simulink subsystem "Subsys_GFormConv_Control"  (R2023b)
settings: Solver=VariableStepAuto  StartTime=0.0  StopTime=10.0  RelTol=1e-3
model mask{S_n=2e6, f_n=50, V_n_phph=690, V_n_grid_phph=20e3, V_n_dc=1380, RL_filter_conv_pu=[ 0.0001 0.05097 ], RC_filter_pu=[ 0.06875 0.04569 ], outputSignal=0, f_sw=5000, sendInfoMessages=0, T_s_ctrl=1e-4, T_s_PWM_meas=1e-4, datatype='double', meas_signals=0, meas_noise_filter=1, f_cutoff_meas=2500, f_cutoff_posseq=20, prot_variant=1, v_dc_max=1.2, v_ac_max=1.1, t_ac_max=0.1, v_ac_maxmax=1.25, t_ac_maxmax=0.1, v_ac_min=0.8, t_ac_min=3, v_ac_minmin=0.45, t_ac_minmin=0.3, f_ac_max=51.5, t_f_ac_max=0.1, f_ac_maxmax=52.5, t_f_ac_maxmax=10, f_ac_min=47.5, t_f_ac_min=0.1, i_ac_max=1.25, OuterCtrlStrategy=0, OuterCtrl_Droop_kP=0.05, OuterCtrl_Droop_kQ=0.1, OuterCtrl_Droop_TQ=0.2, OuterCtrl_ZDroop_kf=0.05, OuterCtrl_ZDroop_kV=0.1, OuterCtrl_ZDroop_kR=0, OuterCtrl_ZDroop_kX=1, OuterCtrl_ZDroop_TV=2, OuterCtrl_Dual_Kp=0.01, OuterCtrl_Dual_Kd=1e-4, OuterCtrl_Dual_kQ=0.1, OuterCtrl_Dual_TQ=0.2, OuterCtrl_VSM_H=0.1, OuterCtrl_VSM_Kd=40, OuterCtrl_VSM_K=20, OuterCtrl_VSM_kQ=0.1, OuterCtrl_VSM_TQ=0.2, L_virt=0, active_damping=1, R_virt_pu=0.2, InnerCtrl_K_p_v_cap=0.8, InnerCtrl_K_i_v_cap=0.5, InnerCtrl_K_p_i_conv=3.3, InnerCtrl_K_i_i_conv=16.5, InnerCtrl_C_ff_v_cap_ctrl=0, InnerCtrl_C_ff_i_conv_ctrl=0, InnerCtrl_K_ff_i=1, InnerCtrl_K_ff_v=1, InnerCtrl_i_conv_max=1, InnerCtrl_v_conv_max=1.3, InnerCtrl_i_lim_type=0}
  mask prompts: S_n "Nominal apparent power [VA]"; f_n "Nominal frequency [Hz]"; V_n_phph "Nominal converter voltage (rms, phase-to-phase) [V]"; V_n_grid_phph "Nominal grid voltage (rms, phase-to-phase) [V]"; V_n_dc "Nominal DC-link voltage [V]"; RL_filter_conv_pu "Impedance of converter-side inductance [ R L ] (pu)"; RC_filter_pu "Impedance of filter capacitor [ R C ] (pu)"; outputSignal "Output signal type (2 = duty cycle (imperix), 1 = switching pulses, 0 = voltage reference (average model))"; f_sw "Switching frequency [Hz]"; sendInfoMessages "Send info messages (1 = enabled, 0 = disabled)"; T_s_ctrl "Controller sample time [s]"; T_s_PWM_meas "PWM and measurements sample time [s]"; datatype "Signal data type"; meas_signals "Measured signals (0 = all signals (tDMSquared simulation), 1 = reduced signals (imperix hardware))"; meas_noise_filter "Low pass to filter measurement noise (1 = enabled, 0 = disabled)"; f_cutoff_meas "Cutoff frequency of low pass filter (measurement noise) [Hz]"; f_cutoff_posseq "Cutoff frequency of low pass filter (positive sequence calculation) [Hz]"; prot_variant "Protection Variant (1 = hardware protection, 2 = tDMSquared warnings only, 3 = deactivated)"; v_dc_max "Maximum DC-link voltage [% nom. value]"; v_ac_max "Maximum AC voltage [% nom. value]"; t_ac_max "Maximum AC voltage timing [s]"; v_ac_maxmax "Upper Maximum AC voltage [% nom. value]"; t_ac_maxmax "Upper Maximum AC voltage timing [s]"; v_ac_min "Upper Minimum AC voltage [% nom. value]"; t_ac_min "Upper Minimum AC voltage timing [s]"; v_ac_minmin "Lower Minimum AC voltage [% nom. value]"; t_ac_minmin "Lower Minimum AC voltage timing [s]"; f_ac_max "Maximum AC frequency [Hz]"; t_f_ac_max "Maximum AC frequency timing [s]"; f_ac_maxmax "Upper Maximum AC frequency [Hz]"; t_f_ac_maxmax "Upper Maximum AC frequency timing [s]"; f_ac_min "Minimum AC frequency [Hz]"; t_f_ac_min "Minimum AC frequency timing [s]"; i_ac_max "Maximum AC current [% nom. value]"; OuterCtrlStrategy "Outer Control Strategy*"; OuterCtrl_Droop_kP "Droop constant kP (df[pu]/dP[pu])"; OuterCtrl_Droop_kQ "Droop constant kQ (dV[pu]/dQ[pu])"; OuterCtrl_Droop_TQ "PT1 time constant QV-loop [s]"; OuterCtrl_ZDroop_kf "Droop constant kf (df/(dP+dQ))"; OuterCtrl_ZDroop_kV "Droop constant kV (dV/(dP+dQ))"; OuterCtrl_ZDroop_kR "R/Z-ratio"; OuterCtrl_ZDroop_kX "X/Z-ratio"; OuterCtrl_ZDroop_TV "PT1 time constant voltage loop [s]"; OuterCtrl_Dual_Kp "Proportional gain [pu]"; OuterCtrl_Dual_Kd "Derivative gain [pu]"; OuterCtrl_Dual_kQ "Droop constant kQ (dV/dQ)"; OuterCtrl_Dual_TQ "PT1 time constant QV-loop T_Q [s]"; OuterCtrl_VSM_H "Virtual inertia [s]"; OuterCtrl_VSM_Kd "Damping constant K_d [pu]"; OuterCtrl_VSM_K "Droop constant K (dT/df) [pu]"; OuterCtrl_VSM_kQ "Droop constant kQ (dV/dQ)"; OuterCtrl_VSM_TQ "PT1 time constant QV-loop T_Q [s]"; L_virt "Virtual output inductance [pu]"; active_damping "Active Damping (1 = enabled, 0 = disabled)"; R_virt_pu "Virtual resistor for active damping (in series with converter-side inductor) [pu]"; InnerCtrl_K_p_v_cap "Voltage controller proportional gain [pu]"; InnerCtrl_K_i_v_cap "Voltage controller integral gain [pu]"; InnerCtrl_K_p_i_conv "Current controller proportional gain [pu]"; InnerCtrl_K_i_i_conv "Current controller integral gain [pu]"; InnerCtrl_C_ff_v_cap_ctrl "Command-feed-forward (voltage controller) (0 = disabled, 1 = enabled)"; InnerCtrl_C_ff_i_conv_ctrl "Command-feed-forward (current controller) (0 = disabled, 1 = enabled)"; InnerCtrl_K_ff_i "Current-feed-forward (voltage controller) (0 = disabled, 1 = enabled)"; InnerCtrl_K_ff_v "Voltage-feed-forward (current controller) (0 = disabled, 1 = enabled)"; InnerCtrl_i_conv_max "Converter current maximum value (limit) [pu]"; InnerCtrl_v_conv_max "Converter voltage maximum value (limit) [pu]"; InnerCtrl_i_lim_type "Coordinate system of current setpoint limiter (0 = dq, 1 = abc)"
libraries: eeTransforms x2, simulink x2, eePwmGeneratorTwoLevel x1
settings Model: Creator=winkens  LastModifiedBy=a.och
settings SolverCC: AlgebraicLoopSolver=TrustRegion
settings OptimizationCC: ReuseModelBlockBuffer=off
settings DebuggingCC: UnconnectedInputMsg=warning  UnconnectedOutputMsg=warning  UnconnectedLineMsg=warning
settings ModelReferenceCC: EnableRefExpFcnMdlSchedulingChecks=on
settings RTWCC: DLArmComputeVersion=19.05

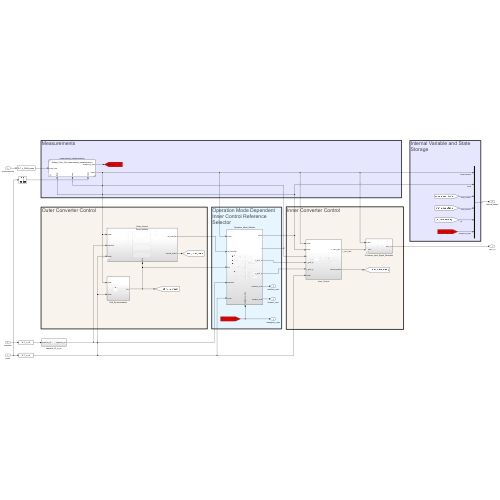
[thumbnail: Simulink's stored preview of the top-level diagram]
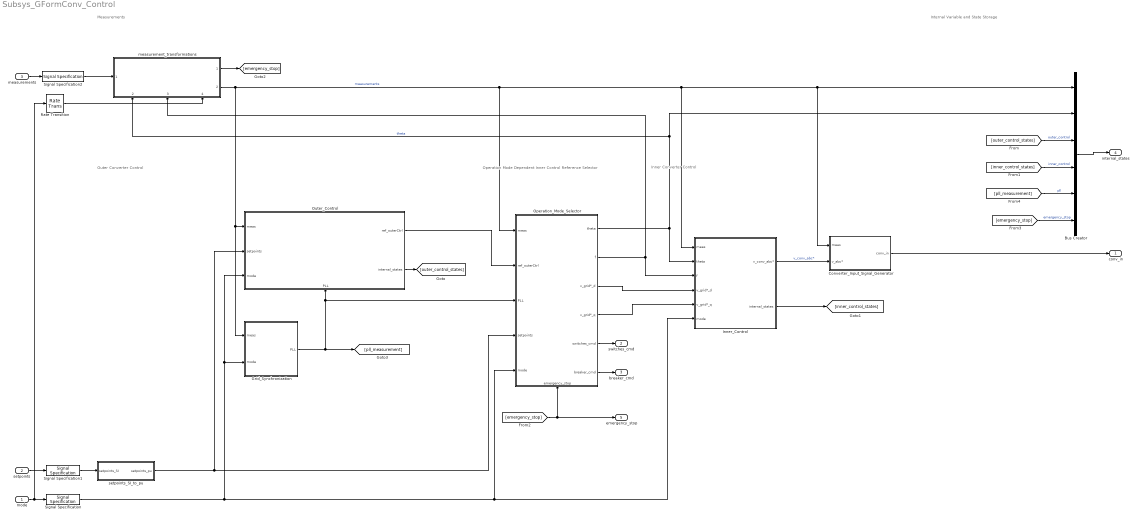
== system Subsys_GFormConv_Control ==
  note: Operation Mode Dependent
      | Inner Control Reference
      | Selector
  note: Outer Converter Control
  note: Internal Variable and State
      | Storage
  note: Inner Converter Control
  note: Measurements
  mode : Inport
  setpoints : Inport  Port=2
  measurements : Inport  Port=3
  Bus Creator : BusCreator  Inputs=6
  Converter_Input_Signal_Generator : Subsystem  Variant=on
  Grid_Synchronization : Subsystem
  Inner_Control : Subsystem
  Operation_Mode_Selector : Subsystem
      settings: PortSchema="{\"entries\":[{\"content\":{\"sides\":[{\"content\":{\"connectorIds\":[\"In1\",\"In2\",\"In3\",\"In4\",\"In5\"]},\"type\":\"ConnectorPlacement.EquallySpacedRectSide\",\"uuid\":\"66bc241c-88d5-476d-bdbe-e179bef52087\"},{\"content\":{\"connectorIds\":[\"Out1\",\"Out2\",\"Out3\",\"Out4\",\"Out5\",\"Out6\"],\"side\":\"RIGHT\"},\"type\":\"ConnectorPlacement.EquallySpacedRectSide\",\"uuid\":\"318c79a0-3cc7-4e7d-956b-e38d7c55976e\"},{\"content\":{\"connectorIds\":[],\"side\":\"TOP\"},\"type\":\"ConnectorPlacement.EquallySpacedRectSide\",\"uuid\":\"dd042cf5-83ab-40ed-a1fe-bca14fe85d10\"},{\"content\":{\"connectorIds\":[\"In6\"],\"side\":\"BOTTOM\"},\"type\":\"ConnectorPlacement.EquallySpacedRectSide\",\"uuid\":\"10d73b36-3b70-4044-8718-174bd2d17802\"},{\"content\":{\"connectorIds\":[],\"side\":\"HIDDEN\"},\"type\":\"ConnectorPlacement.EquallySpacedRectSide\",\"uuid\":\"4c9d2e62-9083-4dbd-9c06-7f98e71bb5f3\"}]},\"type\":\"ConnectorPlacement.EquallySpacedConnector\",\"uuid\":\"f943bfea-1324-4575-985b-fb99fa51a3d8\"}],\"packageUris\":[\"http://schema.mathworks.com/mf0/Connector/R2020b\"],\"version\":\"1.0\"}"
  Outer_Control : Subsystem  Variant=on
      settings: PortSchema="{\"entries\":[{\"content\":{\"sides\":[{\"content\":{\"connectorIds\":[\"In1\",\"In2\",\"In3\"]},\"type\":\"ConnectorPlacement.EquallySpacedRectSide\",\"uuid\":\"253b05e4-806f-4dc0-80d3-d592634157a9\"},{\"content\":{\"connectorIds\":[\"Out1\",\"Out2\"],\"side\":\"RIGHT\"},\"type\":\"ConnectorPlacement.EquallySpacedRectSide\",\"uuid\":\"c3b70f7b-68db-4cd5-a2c2-c4f65ef550a5\"},{\"content\":{\"connectorIds\":[],\"side\":\"TOP\"},\"type\":\"ConnectorPlacement.EquallySpacedRectSide\",\"uuid\":\"830f2dd0-f758-4d50-8b34-5845389ea785\"},{\"content\":{\"connectorIds\":[\"In4\"],\"side\":\"BOTTOM\"},\"type\":\"ConnectorPlacement.EquallySpacedRectSide\",\"uuid\":\"b9313e94-082c-4f29-831f-6939b42f2aae\"},{\"content\":{\"connectorIds\":[],\"side\":\"HIDDEN\"},\"type\":\"ConnectorPlacement.EquallySpacedRectSide\",\"uuid\":\"42ff5aed-1d40-40fc-b6bc-8c88d6312836\"}]},\"type\":\"ConnectorPlacement.EquallySpacedConnector\",\"uuid\":\"adca5aff-478b-45b4-94a3-86875e004fa1\"}],\"packageUris\":[\"http://schema.mathworks.com/mf0/Connector/R2020b\"],\"version\":\"1.0\"}"
  Rate Transition : RateTransition  OutPortSampleTime=T_s_PWM_meas
  Signal Specification : SignalSpecification  SampleTime=T_s_ctrl
  Signal Specification1 : SignalSpecification  SampleTime=T_s_ctrl
  Signal Specification2 : SignalSpecification  SampleTime=T_s_PWM_meas
  measurement_transformations : Subsystem  ReferencedSubsystem=Subsys_Conv_Ctrl_measurement_transformations  S_n=S_n  f_n=f_n  V_n_phph=V_n_phph  V_n_grid_phph=V_n_grid_phph  V_n_dc=V_n_dc  meas_signals=meas_signals  meas_noise_filter=meas_noise_filter  f_cutoff_lowpass=f_cutoff_meas  posseq_calc=0  f_cutoff_posseq=f_cutoff_posseq  prot_variant=prot_variant  v_dc_max=v_dc_max  v_ac_max=v_ac_max  t_ac_max=t_ac_max  v_ac_maxmax=v_ac_maxmax  t_ac_maxmax=t_ac_maxmax  v_ac_min=v_ac_min  t_ac_min=t_ac_min  v_ac_minmin=v_ac_minmin  t_ac_minmin=t_ac_minmin  f_ac_max=f_ac_max  t_f_ac_max=t_f_ac_max  f_ac_maxmax=f_ac_maxmax  t_f_ac_maxmax=t_f_ac_maxmax  f_ac_min=f_ac_min  t_f_ac_min=t_f_ac_min  i_ac_max=i_ac_max  T_s_ctrl=T_s_ctrl  T_s_PWM_meas=T_s_PWM_meas  datatype=datatype
      settings: PortSchema="{\"entries\":[{\"content\":{\"sides\":[{\"content\":{\"connectorIds\":[\"In1\"]},\"type\":\"ConnectorPlacement.EquallySpacedRectSide\",\"uuid\":\"ec41b0e2-5656-4860-9e39-a664af2bd5a5\"},{\"content\":{\"connectorIds\":[\"Out1\",\"Out2\"],\"side\":\"RIGHT\"},\"type\":\"ConnectorPlacement.EquallySpacedRectSide\",\"uuid\":\"80e01e50-a82e-48c2-876d-2e84cdeaf8f0\"},{\"content\":{\"side\":\"TOP\"},\"type\":\"ConnectorPlacement.EquallySpacedRectSide\",\"uuid\":\"663ee62b-f6cc-4583-9600-029eedfe0a7c\"},{\"content\":{\"connectorIds\":[\"In2\",\"In3\",\"In4\"],\"side\":\"BOTTOM\"},\"type\":\"ConnectorPlacement.EquallySpacedRectSide\",\"uuid\":\"c2907c22-84a2-4ef4-81a7-f2773dfe6a2a\"},{\"content\":{\"side\":\"HIDDEN\"},\"type\":\"ConnectorPlacement.EquallySpacedRectSide\",\"uuid\":\"af4de394-2758-4e50-9887-b7deaef1f38c\"}]},\"type\":\"ConnectorPlacement.EquallySpacedConnector\",\"uuid\":\"1362d2e6-f83a-419a-8b0e-95b4449907fb\"}],\"packageUris\":[\"http://schema.mathworks.com/mf0/Connector/R2020b\"],\"version\":\"1.0\"}"
  setpoints_SI_to_pu : Subsystem
  conv_in : Outport
  switches_cmd : Outport  Port=2
  breaker_cmd : Outport  Port=3
  internal_states : Outport  Port=4
  emergency_stop : Outport  Port=5
  wires:
  Rate Transition/1 -> measurement_transformations/4
  Operation_Mode_Selector/2(f) -> measurement_transformations/3, Inner_Control/3(f)
  setpoints/1 -> Signal Specification1/1
  Inner_Control/1(v_conv_abc*) -> Converter_Input_Signal_Generator/2(v_abc*)  "v_conv_abc*"
  Inner_Control/2(internal_states) -> [inner_control_states]
  [outer_control_states] -> Bus Creator/3  "outer_control"
  [inner_control_states] -> Bus Creator/4  "inner_control"
  Bus Creator/1 -> internal_states/1
  Outer_Control/2(internal_states) -> [outer_control_states]
  mode/1 -> Signal Specification/1, Rate Transition/1
  Operation_Mode_Selector/3(v_grid*_d) -> Inner_Control/4(v_grid*_d)
  Operation_Mode_Selector/1(theta) -> Inner_Control/2(theta), Bus Creator/2, measurement_transformations/2  "theta"
  Outer_Control/1(ref_outerCtrl) -> Operation_Mode_Selector/2(ref_outerCtrl)
  Operation_Mode_Selector/5(switches_cmd) -> switches_cmd/1
  Operation_Mode_Selector/6(breaker_cmd) -> breaker_cmd/1
  Converter_Input_Signal_Generator/1(conv_in) -> conv_in/1
  setpoints_SI_to_pu/1(setpoints_pu) -> Outer_Control/2(setpoints), Operation_Mode_Selector/4(setpoints)
  Grid_Synchronization/1(PLL) -> [pll_measurement], Operation_Mode_Selector/3(PLL), Outer_Control/4(PLL)
  measurement_transformations/2 -> Outer_Control/1(meas), Grid_Synchronization/1(meas), Converter_Input_Signal_Generator/1(meas), Bus Creator/1, Inner_Control/1(meas), Operation_Mode_Selector/1(meas)  "measurements"
  measurements/1 -> Signal Specification2/1
  measurement_transformations/1 -> [emergency_stop]
  [emergency_stop] -> emergency_stop/1, Operation_Mode_Selector/6(emergency_stop)
  Signal Specification/1 -> Inner_Control/6(mode), Operation_Mode_Selector/5(mode), Grid_Synchronization/2(mode), Outer_Control/3(mode)
  Signal Specification1/1 -> setpoints_SI_to_pu/1(setpoints_SI)
  Signal Specification2/1 -> measurement_transformations/1
  Operation_Mode_Selector/4(v_grid*_q) -> Inner_Control/5(v_grid*_q)
  [emergency_stop] -> Bus Creator/6  "emergency_stop"
  [pll_measurement] -> Bus Creator/5  "pll"

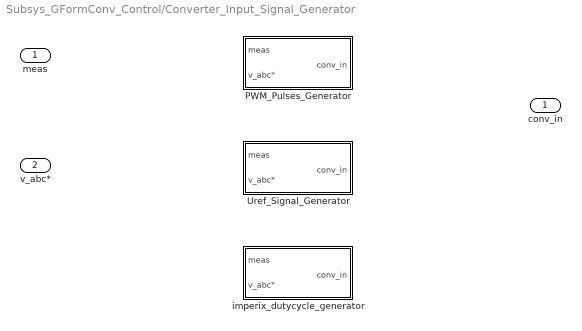
== system Subsys_GFormConv_Control/Converter_Input_Signal_Generator ==
  meas : Inport
  v_abc* : Inport  Port=2
  PWM_Pulses_Generator : Subsystem  VariantControl=outputSignal == 1
  Uref_Signal_Generator : Subsystem  VariantControl=(default)
  imperix_dutycycle_generator : Subsystem  VariantControl=outputSignal == 2
  conv_in : Outport

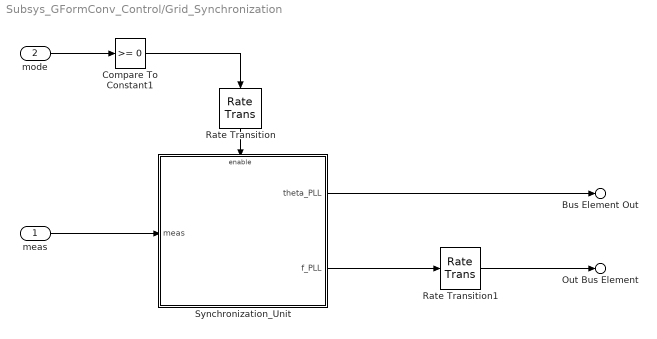
== system Subsys_GFormConv_Control/Grid_Synchronization ==
  meas : Inport
  mode : Inport  Port=2
  Compare To Constant1 : simulink/Logic and Bit Operations/Compare To Constant  relop=>=  const=0  OutDataTypeStr=boolean
  Rate Transition : RateTransition  Deterministic=off  OutPortSampleTime=T_s_PWM_meas
  Rate Transition1 : RateTransition  Deterministic=off  OutPortSampleTime=T_s_ctrl
  Synchronization_Unit : Subsystem
  Bus Element Out : Outport  PortName=PLL  Element=theta_PLL
  Out Bus Element : Outport  PortName=PLL  Element=f_PLL
  wires:
  meas/1 -> Synchronization_Unit/1(meas)
  mode/1 -> Compare To Constant1/1
  Compare To Constant1/1 -> Rate Transition/1
  Synchronization_Unit/1(theta_PLL) -> Bus Element Out/1
  Synchronization_Unit/2(f_PLL) -> Rate Transition1/1
  Rate Transition/1 -> Synchronization_Unit/Enable
  Rate Transition1/1 -> Out Bus Element/1

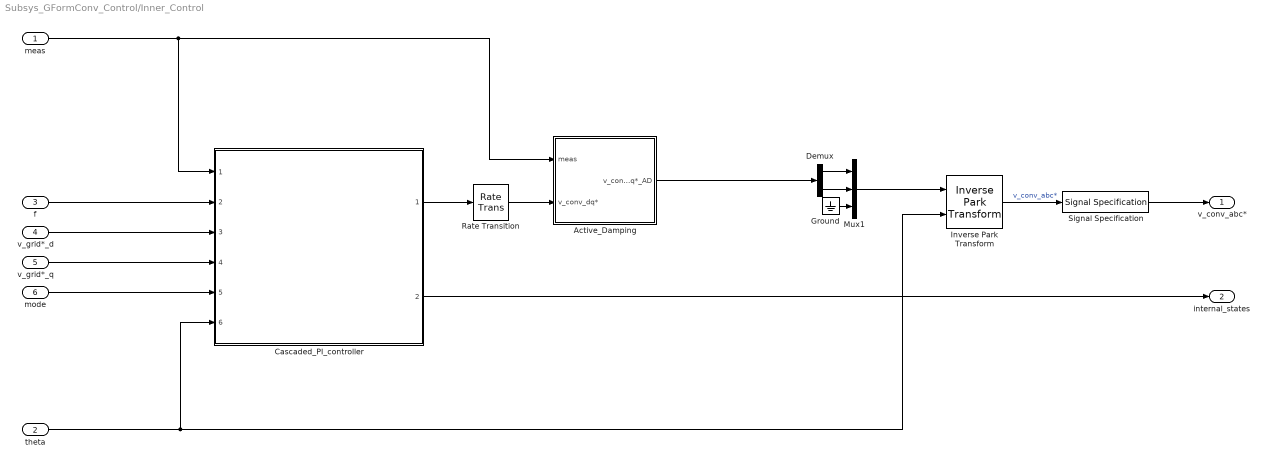
== system Subsys_GFormConv_Control/Inner_Control ==
  meas : Inport
  theta : Inport  Port=2  PortDimensions=1
  f : Inport  Port=3  PortDimensions=1
  v_grid*_d : Inport  Port=4  PortDimensions=1
  v_grid*_q : Inport  Port=5  PortDimensions=1
  mode : Inport  Port=6  PortDimensions=1
  Active_Damping : Subsystem  Variant=on  VariantControl=Choice
  Cascaded_PI_controller : Subsystem  ReferencedSubsystem=Subsys_GFormConv_InnerCtrl_cascadedPI  f_n=f_n  L_filter_conv_pu=RL_filter_conv_pu  C_filter_pu=RC_filter_pu  send_info_messages=sendInfoMessages  K_p_V_cap_controller=InnerCtrl_K_p_v_cap  K_i_V_cap_controller=InnerCtrl_K_i_v_cap  K_p_I_conv_controller=InnerCtrl_K_p_i_conv  K_i_I_conv_controller=InnerCtrl_K_i_i_conv  Cff_V_cap_ctrl=InnerCtrl_C_ff_v_cap_ctrl  Cff_I_conv_ctrl=InnerCtrl_C_ff_i_conv_ctrl  K_ff_I_grid=InnerCtrl_K_ff_i  K_ff_V_cap=InnerCtrl_K_ff_v  i_conv_limit=InnerCtrl_i_conv_max  v_conv_limit=InnerCtrl_v_conv_max  i_lim_type=InnerCtrl_i_lim_type  T_s_ctrl=T_s_ctrl  T_s_PWM_meas=T_s_PWM_meas  datatype=datatype
  Demux : Demux  Outputs=2
  Ground : Ground
  Inverse Park Transform : eeTransforms/Inverse Park Transform  AxisAlignment=D-axis  PowerInvariant=off
  Mux1 : Mux  Inputs=3
  Rate Transition : RateTransition  Deterministic=off  OutPortSampleTime=T_s_PWM_meas
  Signal Specification : SignalSpecification  SampleTime=T_s_PWM_meas
  v_conv_abc* : Outport  PortDimensions=3
  internal_states : Outport  Port=2
  wires:
  meas/1 -> Active_Damping/1(meas), Cascaded_PI_controller/1
  f/1 -> Cascaded_PI_controller/2
  v_grid*_d/1 -> Cascaded_PI_controller/3
  mode/1 -> Cascaded_PI_controller/5
  Cascaded_PI_controller/2 -> internal_states/1
  Mux1/1 -> Inverse Park Transform/1
  Ground/1 -> Mux1/3
  Demux/2 -> Mux1/2
  Demux/1 -> Mux1/1
  theta/1 -> Cascaded_PI_controller/6, Inverse Park Transform/2
  Cascaded_PI_controller/1 -> Rate Transition/1
  Inverse Park Transform/1 -> Signal Specification/1  "v_conv_abc*"
  Active_Damping/1(v_conv_dq*_AD) -> Demux/1
  Signal Specification/1 -> v_conv_abc*/1
  Rate Transition/1 -> Active_Damping/2(v_conv_dq*)
  v_grid*_q/1 -> Cascaded_PI_controller/4

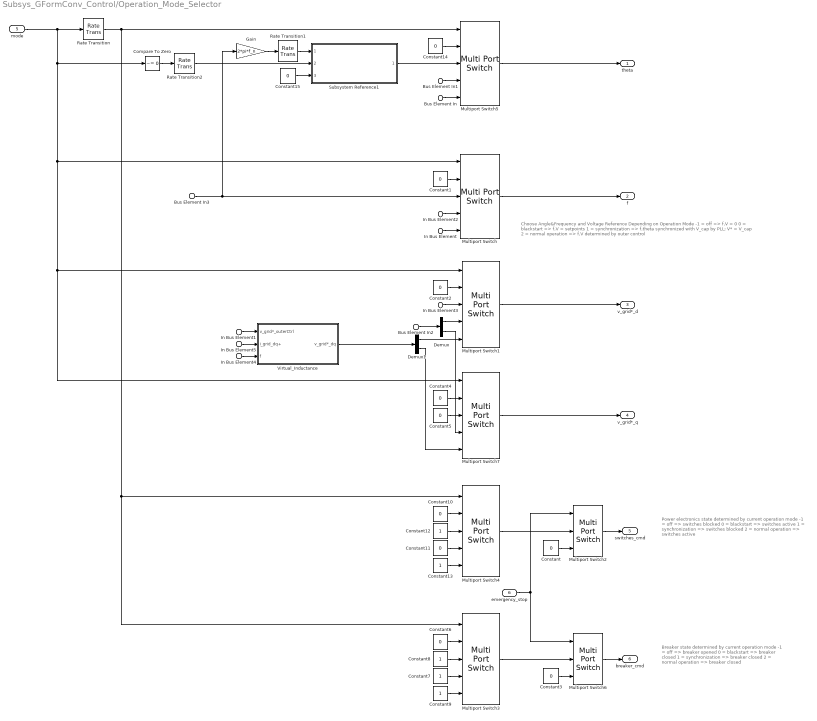
== system Subsys_GFormConv_Control/Operation_Mode_Selector ==
  note: Choose Angle&Frequency and Voltage Reference Depending on Operation Mode
      | -1 = off => f,V = 0
      | 0 = blackstart => f,V = setpoints
      | 1 = synchronization => f,theta synchronized with V_cap by PLL; V* = V_cap
      | 2 = normal operation => f,V determined by outer control
  note: Breaker state determined by current operation mode
      | -1 = off => breaker opened
      | 0  = blackstart => breaker closed
      | 1  = synchronization => breaker closed
      | 2  = normal operation => breaker closed
  note: Power electronics state determined by current operation mode
      | -1 = off => switches blocked
      | 0  = blackstart => switches active
      | 1  = synchronization => switches blocked
      | 2  = normal operation => switches active
  Bus Element In2 : Inport  PortName=meas  Element=dq+.v_cap_dq+
  In Bus Element5 : Inport  PortName=meas  Element=dq+.i_grid_dq+
  Bus Element In : Inport  Port=2  PortName=ref_outerCtrl  Element=theta
  In Bus Element : Inport  Port=2  PortName=ref_outerCtrl  Element=f
  In Bus Element4 : Inport  Port=2  PortName=ref_outerCtrl  Element=f
  In Bus Element1 : Inport  Port=2  PortName=ref_outerCtrl  Element=v_grid*
  Bus Element In1 : Inport  Port=3  PortName=PLL  Element=theta_PLL
  In Bus Element2 : Inport  Port=3  PortName=PLL  Element=f_PLL
  Bus Element In3 : Inport  Port=4  PortName=setpoints  Element=f_set_pu
  In Bus Element3 : Inport  Port=4  PortName=setpoints  Element=v_set
  mode : Inport  Port=5
  emergency_stop : Inport  Port=6
  Compare To Zero : simulink/Logic and Bit Operations/Compare To Zero  relop=~=  OutDataTypeStr=boolean
  Constant{,3,6,10..11} (5 alike) : Constant  Value=0  OutDataTypeStr=boolean
  Constant{1..2,4..5,14} (5 alike) : Constant  Value=0  OutDataTypeStr=datatype
  Constant{7..9,12..13} (5 alike) : Constant  OutDataTypeStr=boolean
  Constant15 : Constant  Value=0
  Demux : Demux  Outputs=2
  Demux1 : Demux  Outputs=2
  Gain : Gain  Gain=2*pi*f_n
  Multiport Switch{,1,3..5,7} (6 alike) : MultiPortSwitch  DataPortOrder=Specify indices  DataPortIndices={-1,0,1,2}  SaturateOnIntegerOverflow=off  InputSameDT=off
  Multiport Switch2 : MultiPortSwitch  DataPortOrder=Specify indices  DataPortIndices={0,1}  SaturateOnIntegerOverflow=off  InputSameDT=off
  Multiport Switch6 : MultiPortSwitch  DataPortOrder=Specify indices  DataPortIndices={0,1}  SaturateOnIntegerOverflow=off  InputSameDT=off
  Rate Transition : RateTransition  Deterministic=off  OutPortSampleTime=T_s_PWM_meas
  Rate Transition1 : RateTransition  Deterministic=off  OutPortSampleTime=T_s_PWM_meas
  Rate Transition2 : RateTransition  Deterministic=off  OutPortSampleTime=T_s_PWM_meas
  Subsystem Reference1 : Subsystem  ReferencedSubsystem=Integrator_discrete_wrapped_state  WrappedStateUpperValue=2*pi  WrappedStateLowerValue=0  x_0=0  T_s=T_s_PWM_meas
  Virtual_Inductance : Subsystem
  theta : Outport
  f : Outport  Port=2
  v_grid*_d : Outport  Port=3
  v_grid*_q : Outport  Port=4
  switches_cmd : Outport  Port=5
  breaker_cmd : Outport  Port=6
  wires:
  Gain/1 -> Rate Transition1/1
  Bus Element In1/1 -> Multiport Switch5/4
  In Bus Element2/1 -> Multiport Switch/4
  Demux/1 -> Multiport Switch1/4
  In Bus Element3/1 -> Multiport Switch1/3
  Bus Element In3/1 -> Multiport Switch/3, Gain/1
  Constant2/1 -> Multiport Switch1/2
  In Bus Element/1 -> Multiport Switch/5
  Constant1/1 -> Multiport Switch/2
  Multiport Switch1/1 -> v_grid*_d/1
  Multiport Switch/1 -> f/1
  Constant7/1 -> Multiport Switch3/4
  Constant6/1 -> Multiport Switch3/2
  Constant10/1 -> Multiport Switch4/2
  Constant8/1 -> Multiport Switch3/3
  Constant12/1 -> Multiport Switch4/3
  Constant13/1 -> Multiport Switch4/5
  Constant9/1 -> Multiport Switch3/5
  Constant11/1 -> Multiport Switch4/4
  mode/1 -> Rate Transition/1, Compare To Zero/1, Multiport Switch/1, Multiport Switch7/1, Multiport Switch1/1
  Bus Element In/1 -> Multiport Switch5/5
  Demux/2 -> Multiport Switch7/4
  Multiport Switch5/1 -> theta/1
  Constant14/1 -> Multiport Switch5/2
  Constant15/1 -> Subsystem Reference1/3
  Compare To Zero/1 -> Rate Transition2/1
  Subsystem Reference1/1 -> Multiport Switch5/3
  emergency_stop/1 -> Multiport Switch6/1, Multiport Switch2/1
  Multiport Switch2/1 -> switches_cmd/1
  Multiport Switch6/1 -> breaker_cmd/1
  Multiport Switch3/1 -> Multiport Switch6/2
  Multiport Switch4/1 -> Multiport Switch2/2
  Constant/1 -> Multiport Switch2/3
  Constant3/1 -> Multiport Switch6/3
  Bus Element In2/1 -> Demux/1
  Rate Transition/1 -> Multiport Switch3/1, Multiport Switch4/1, Multiport Switch5/1
  Rate Transition1/1 -> Subsystem Reference1/1
  Rate Transition2/1 -> Subsystem Reference1/2
  Multiport Switch7/1 -> v_grid*_q/1
  Constant5/1 -> Multiport Switch7/3
  Constant4/1 -> Multiport Switch7/2
  Demux1/1 -> Multiport Switch1/5
  Virtual_Inductance/1(v_grid*_dq) -> Demux1/1
  Demux1/2 -> Multiport Switch7/5
  In Bus Element1/1 -> Virtual_Inductance/1(v_grid*_outerCtrl)
  In Bus Element4/1 -> Virtual_Inductance/3(f)
  In Bus Element5/1 -> Virtual_Inductance/2(i_grid_dq+)

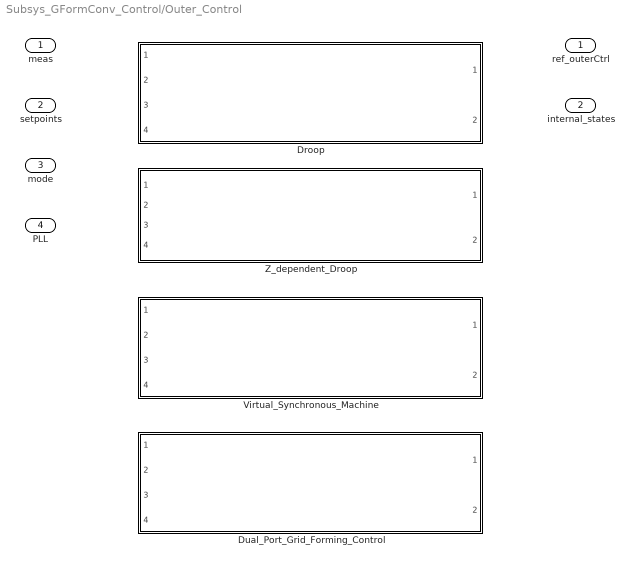
== system Subsys_GFormConv_Control/Outer_Control ==
  meas : Inport
  setpoints : Inport  Port=2
  mode : Inport  Port=3
  PLL : Inport  Port=4
  Droop : Subsystem  VariantControl=(default)  ReferencedSubsystem=Subsys_GFormConv_OuterCtrl_Droop  f_n=f_n  s_droop_Pf=OuterCtrl_Droop_kP  s_droop_QV=OuterCtrl_Droop_kQ  T_Q=OuterCtrl_Droop_TQ  T_s_ctrl=T_s_ctrl  T_s_PWM_meas=T_s_PWM_meas
  Dual_Port_Grid_Forming_Control : Subsystem  VariantControl=OuterCtrlStrategy == 3  ReferencedSubsystem=Subsys_GFormConv_OuterCtrl_Dual_Port  f_n=f_n  K_p=OuterCtrl_Dual_Kp  K_d=OuterCtrl_Dual_Kd  s_droop_QV=OuterCtrl_Dual_kQ  T_Q=OuterCtrl_Dual_TQ  T_s_ctrl=T_s_ctrl  T_s_PWM_meas=T_s_PWM_meas
  Virtual_Synchronous_Machine : Subsystem  VariantControl=OuterCtrlStrategy == 2  ReferencedSubsystem=Subsys_GFormConv_OuterCtrl_VSM  f_n=f_n  H=OuterCtrl_VSM_H  K_d=OuterCtrl_VSM_Kd  K=OuterCtrl_VSM_K  s_droop_QV=OuterCtrl_VSM_kQ  T_Q=OuterCtrl_VSM_TQ  T_s_ctrl=T_s_ctrl  T_s_PWM_meas=T_s_PWM_meas
  Z_dependent_Droop : Subsystem  VariantControl=OuterCtrlStrategy == 1  ReferencedSubsystem=Subsys_GFormConv_OuterCtrl_ZDepDroop  f_n=f_n  k_f=OuterCtrl_ZDroop_kf  k_V=OuterCtrl_ZDroop_kV  k_R=OuterCtrl_ZDroop_kR  k_X=OuterCtrl_ZDroop_kX  T_V=OuterCtrl_ZDroop_TV  T_s_ctrl=T_s_ctrl  T_s_PWM_meas=T_s_PWM_meas
  ref_outerCtrl : Outport
  internal_states : Outport  Port=2

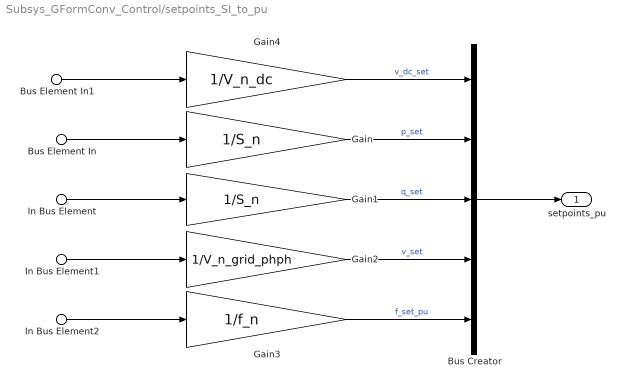
== system Subsys_GFormConv_Control/setpoints_SI_to_pu ==
  Bus Element In : Inport  PortName=setpoints_SI  Element=P_set
  In Bus Element : Inport  PortName=setpoints_SI  Element=Q_set
  In Bus Element1 : Inport  PortName=setpoints_SI  Element=V_set_phph
  In Bus Element2 : Inport  PortName=setpoints_SI  Element=f_set
  Bus Element In1 : Inport  PortName=setpoints_SI  Element=V_dc_set
  Bus Creator : BusCreator  Inputs=5
  Gain : Gain  Gain=1/S_n
  Gain1 : Gain  Gain=1/S_n
  Gain2 : Gain  Gain=1/V_n_grid_phph
  Gain3 : Gain  Gain=1/f_n
  Gain4 : Gain  Gain=1/V_n_dc
  setpoints_pu : Outport
  wires:
  Bus Creator/1 -> setpoints_pu/1
  Gain3/1 -> Bus Creator/5  "f_set_pu"
  Gain2/1 -> Bus Creator/4  "v_set"
  Gain1/1 -> Bus Creator/3  "q_set"
  Gain/1 -> Bus Creator/2  "p_set"
  In Bus Element2/1 -> Gain3/1
  In Bus Element1/1 -> Gain2/1
  In Bus Element/1 -> Gain1/1
  Bus Element In/1 -> Gain/1
  Bus Element In1/1 -> Gain4/1
  Gain4/1 -> Bus Creator/1  "v_dc_set"

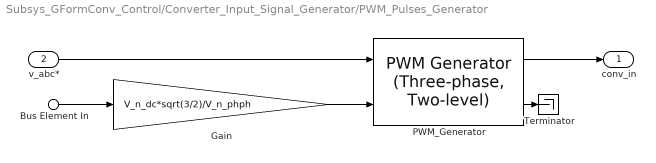
== system Subsys_GFormConv_Control/Converter_Input_Signal_Generator/PWM_Pulses_Generator ==
  Bus Element In : Inport  PortName=meas  Element=v_dc
  v_abc* : Inport  Port=2
  Gain : Gain  Gain=V_n_dc*sqrt(3/2)/V_n_phph
  PWM_Generator : eePwmGeneratorTwoLevel/PWM Generator (Three-phase, Two-level)  PWMMode=Continuous PWM (CPWM)  CPWMMode=SPWM: sinusoidal PWM  DPWMMode=60 DPWM: 60 degree discontinuous PWM  fsw=f_sw  Ts=T_s_PWM_meas(1)
  Terminator : Terminator
  conv_in : Outport
  wires:
  Bus Element In/1 -> Gain/1
  v_abc*/1 -> PWM_Generator/1
  PWM_Generator/1 -> conv_in/1
  PWM_Generator/2 -> Terminator/1
  Gain/1 -> PWM_Generator/2

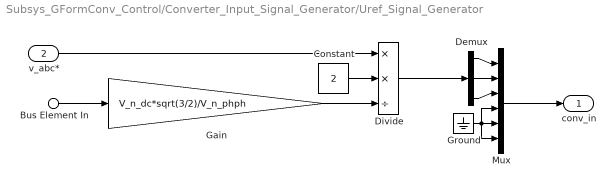
== system Subsys_GFormConv_Control/Converter_Input_Signal_Generator/Uref_Signal_Generator ==
  Bus Element In : Inport  PortName=meas  Element=v_dc
  v_abc* : Inport  Port=2
  Constant : Constant  Value=2  OutDataTypeStr=datatype
  Demux : Demux  Outputs=3
  Divide : Product  Inputs=**/
  Gain : Gain  Gain=V_n_dc*sqrt(3/2)/V_n_phph
  Ground : Ground
  Mux : Mux  Inputs=6
  conv_in : Outport
  wires:
  v_abc*/1 -> Divide/1
  Bus Element In/1 -> Gain/1
  Constant/1 -> Divide/2
  Demux/1 -> Mux/1
  Demux/2 -> Mux/2
  Demux/3 -> Mux/3
  Ground/1 -> Mux/6, Mux/4, Mux/5
  Mux/1 -> conv_in/1
  Divide/1 -> Demux/1
  Gain/1 -> Divide/3

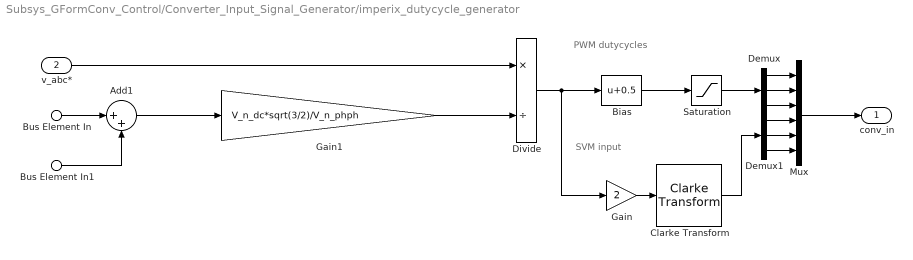
== system Subsys_GFormConv_Control/Converter_Input_Signal_Generator/imperix_dutycycle_generator ==
  note: SVM input
  note: PWM dutycycles
  Bus Element In : Inport  PortName=meas  Element=v_dc_low
  Bus Element In1 : Inport  PortName=meas  Element=v_dc_up
  v_abc* : Inport  Port=2
  Add1 : Sum  Inputs=|++
  Bias : Bias  Bias=0.5  SaturateOnIntegerOverflow=off
  Clarke Transform : eeTransforms/Clarke Transform  PowerInvariant=off
  Demux : Demux  Outputs=3
  Demux1 : Demux  Outputs=3
  Divide : Product  Inputs=*/
  Gain : Gain  Gain=2
  Gain1 : Gain  Gain=V_n_dc*sqrt(3/2)/V_n_phph
  Mux : Mux  Inputs=6
  Saturation : Saturate  UpperLimit=1  LowerLimit=0
  conv_in : Outport
  wires:
  Bus Element In/1 -> Add1/1
  Demux/1 -> Mux/1
  Demux/2 -> Mux/2
  Demux/3 -> Mux/3
  Mux/1 -> conv_in/1
  Divide/1 -> Gain/1, Bias/1
  v_abc*/1 -> Divide/1
  Bus Element In1/1 -> Add1/2
  Saturation/1 -> Demux/1
  Bias/1 -> Saturation/1
  Demux1/1 -> Mux/4
  Demux1/2 -> Mux/5
  Demux1/3 -> Mux/6
  Clarke Transform/1 -> Demux1/1
  Add1/1 -> Gain1/1
  Gain/1 -> Clarke Transform/1
  Gain1/1 -> Divide/2

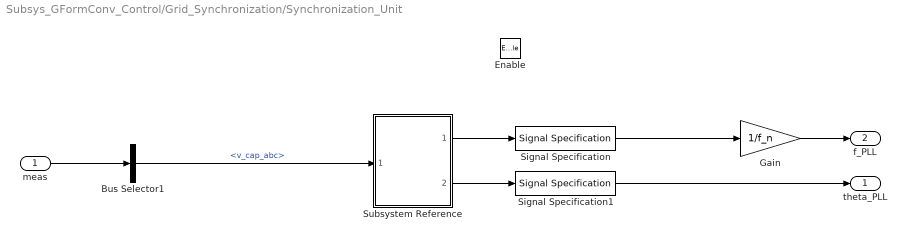
== system Subsys_GFormConv_Control/Grid_Synchronization/Synchronization_Unit ==
  meas : Inport
  Enable : EnablePort
  Bus Selector1 : BusSelector  OutputSignals=abc.v_cap_abc
  Gain : Gain  Gain=1/f_n
  Signal Specification : SignalSpecification  SampleTime=T_s_PWM_meas
  Signal Specification1 : SignalSpecification  SampleTime=T_s_PWM_meas
  Subsystem Reference : Subsystem  ReferencedSubsystem=PLL  f_n=f_n  K_p=180  K_i=3200  df_max=f_n  f_c=25  theta_feedback=1  T_s=T_s_PWM_meas  datatype=datatype
  theta_PLL : Outport
  f_PLL : Outport  Port=2
  wires:
  Gain/1 -> f_PLL/1
  Bus Selector1/1 -> Subsystem Reference/1  "<v_cap_abc>"
  meas/1 -> Bus Selector1/1
  Signal Specification1/1 -> theta_PLL/1
  Signal Specification/1 -> Gain/1
  Subsystem Reference/1 -> Signal Specification/1
  Subsystem Reference/2 -> Signal Specification1/1

== system Subsys_GFormConv_Control/Inner_Control/Active_Damping ==
  meas : Inport
  v_conv_dq* : Inport  Port=2
  No_Damping : Subsystem  VariantControl=(default)
  Virtual_Resistor : Subsystem  VariantControl=active_damping > 0.5
  v_conv_dq*_AD : Outport

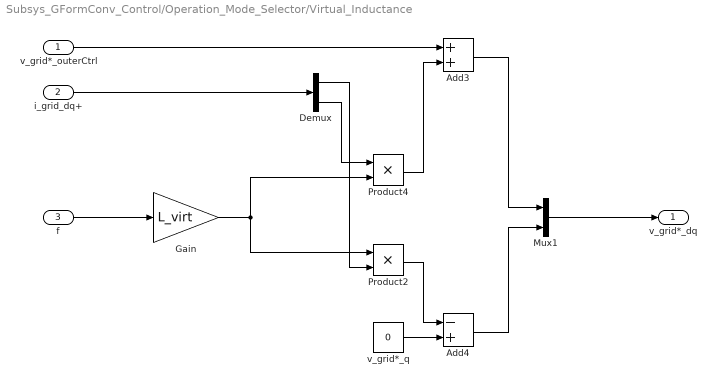
== system Subsys_GFormConv_Control/Operation_Mode_Selector/Virtual_Inductance ==
  v_grid*_outerCtrl : Inport
  i_grid_dq+ : Inport  Port=2
  f : Inport  Port=3
  Add3 : Sum
  Add4 : Sum  Inputs=-+
  Demux : Demux  Outputs=2
  Gain : Gain  Gain=L_virt
  Mux1 : Mux  Inputs=2
  Product2 : Product
  Product4 : Product
  v_grid*_q : Constant  Value=0  OutDataTypeStr=datatype  LockScale=on
  v_grid*_dq : Outport
  wires:
  f/1 -> Gain/1
  Demux/2 -> Product4/1
  Demux/1 -> Product2/2
  Gain/1 -> Product4/2, Product2/1
  Product2/1 -> Add4/1
  Product4/1 -> Add3/2
  v_grid*_q/1 -> Add4/2
  v_grid*_outerCtrl/1 -> Add3/1
  Mux1/1 -> v_grid*_dq/1
  Add4/1 -> Mux1/2
  Add3/1 -> Mux1/1
  i_grid_dq+/1 -> Demux/1

== system Subsys_GFormConv_Control/Inner_Control/Active_Damping/No_Damping ==
  meas : Inport
  v_conv_dq* : Inport  Port=2
  Terminator : Terminator
  v_conv_dq*_AD : Outport
  wires:
  meas/1 -> Terminator/1
  v_conv_dq*/1 -> v_conv_dq*_AD/1

== system Subsys_GFormConv_Control/Inner_Control/Active_Damping/Virtual_Resistor ==
  Bus Element In : Inport  PortName=meas  Element=dq0.i_conv_dq0
  v_conv_dq* : Inport  Port=2
  AD Resistor : Gain  Gain=R_virt_pu
  Add : Sum  Inputs=-+|
  Selector : Selector  InputPortWidth=3  IndexOptions=Index vector (dialog)  Indices=[1 2]  OutputSizes=1
  v_conv_dq*_AD : Outport
  wires:
  AD Resistor/1 -> Add/1
  Add/1 -> v_conv_dq*_AD/1
  v_conv_dq*/1 -> Add/2
  Selector/1 -> AD Resistor/1
  Bus Element In/1 -> Selector/1
